simulink model "sign_detector"  (R2026b)
settings: Solver=FixedStepDiscrete  StopTime=5  FixedStep=0.025  EnableMultiTasking=on
values from neighbouring files (symbols this model uses):
  CAN_PERIOD = 0.1    [sign_detector.sldd]
  INFER_PERIOD = 0.05    [sign_detector.sldd]
libraries: raspberrypiAVlib x1
settings Model: DataDictionary=sign_detector.sldd  Creator=don  LastModifiedBy=don
settings SolverCC: PositivePriorityOrder=on
settings OptimizationCC: DifferentSizesBufferReuse=on  EfficientFloat2IntCast=on  EfficientTunableParamExpr=on  EnhancedBackFolding=on  LifeSpan=Inf  MaxStackSize=200000  OptimizationCustomize=off  OptimizeBlockOrder=speed  PassReuseOutputArgsAs=Individual arguments  UseDivisionForNetSlopeComputation=on
settings DebuggingCC: AlgebraicLoopMsg=error  ArtificialAlgebraicLoopMsg=error  AssertControl=DisableAll  BlockPriorityViolationMsg=error  BusObjectLabelMismatch=error  CheckMatrixSingularityMsg=error  InheritedTsInSrcMsg=error  IntegerOverflowMsg=error  IntegerSaturationMsg=error  ModelReferenceDataLoggingMessage=error  ModelReferenceIOMismatchMessage=error  NonBusSignalsTreatedAsBus=error  ParameterPrecisionLossMsg=error  ParameterTunabilityLossMsg=error  ParameterUnderflowMsg=error  ReadBeforeWriteMsg=EnableAllAsError  RootOutportRequireBusObject=error  SFcnCompatibilityMsg=error  SaveWithDisabledLinksMsg=error  SaveWithParameterizedLinksMsg=error  SigSpecEnsureSampleTimeMsg=error  SignalInfNanChecking=error  SignalLabelMismatchMsg=error  SignalRangeChecking=error  SolverPrmCheckMsg=error  StateNameClashWarn=warning  StrictBusMsg=ErrorOnBusTreatedAsVector  TasksWithSamePriorityMsg=error  UnconnectedInputMsg=error  UnconnectedLineMsg=error  UnconnectedOutputMsg=error  UnderSpecifiedDataTypeMsg=error  UniqueDataStoreMsg=error  UnknownTsInhSupMsg=error  UnnecessaryDatatypeConvMsg=warning  VariantConditionMismatch=error  VectorMatrixConversionMsg=error  WriteAfterReadMsg=EnableAllAsError  WriteAfterWriteMsg=EnableAllAsError
settings HardwareCC: ProdHWDeviceType=ARM Compatible->ARM Cortex-A (64-bit)  ProdLargestAtomicFloat=Double  ProdLargestAtomicInteger=LongLong  ProdLongLongMode=on
settings ModelReferenceCC: ModelReferenceNumInstancesAllowed=Single
settings SFSimCC: EnableRuntimeRecursion=off  MATLABDynamicMemAlloc=off
settings RTWCC: BuildConfiguration=Faster Runs  CustomInitializer=ncnn_infer_preload();  Description=Embedded Coder  HardwareBoard=Raspberry Pi (64bit)  PostCodeGenCommand=codertarget.postCodeGenHookCommand(h); pi_postcodegen(buildInfo, string.empty)  SystemTargetFile=ert.tlc  TLCOptions="-aInlineSetEventsForThisBaseRateFcn=TLC_FALSE -aSuppressMultiTaskScheduler=TLC_FALSE  -aRateBasedStepFcn=0"  TargetLang=C++  TemplateMakefile=ert_default_tmf  Toolchain=GNU GCC RPIUtils
settings RTWCC: CustomHeaderCode=|
  | #include <time.h>
  | /* clock_now (Clock Infer, Clock CAN 블록): 단조 시계 [초], Pi 생성 코드에서만 씀 */
  | static inline double mono_time_sec(void)
  | {
  |     struct timespec ts;
  |     clock_gettime(CLOCK_MONOTONIC, &ts);
  |     return (double)ts.tv_sec + (double)ts.tv_nsec * 1e-9;
  | }
  | 
  | /* ncnn_infer.cpp (unit_recognize): 주기 태스크 시작 전에 모델 파일을 읽음 (HIL: 시작 직후 송신 간격 지연 해결) */
  | #ifdef __cplusplus
  | extern "C"
  | #endif
  | int ncnn_infer_preload(void);
settings CodeAppCC: ForceParamTrailComments=on  IgnoreCustomStorageClasses=off  InsertBlockDesc=on  MATLABFcnDesc=on  MATLABSourceComments=on  OperatorAnnotations=on  ReqsInCode=on  SFDataObjDesc=on  SimulinkDataObjDesc=on  StateflowObjectComments=on
settings ERTTargetCC: CastingMode=Standards  CombineSignalStateStructs=on  EnableSignedLeftShifts=off  EnableSignedRightShifts=off  ExtModeIntrfLevel=Level2 - Open  ExtModeMexFile=ext_xcp  ExtModeStaticAlloc=on  GenerateSharedConstants=off  ParenthesesLevel=Standards  PreserveExpressionOrder=on  SubcomponentCodeInterfacePackaging=Nonreusable function  SupportNonFinite=off  SupportVariableSizeSignals=on  SuppressErrorStatus=on  TargetLangStandard=C++11 (ISO)  UtilityFuncGeneration=Shared location

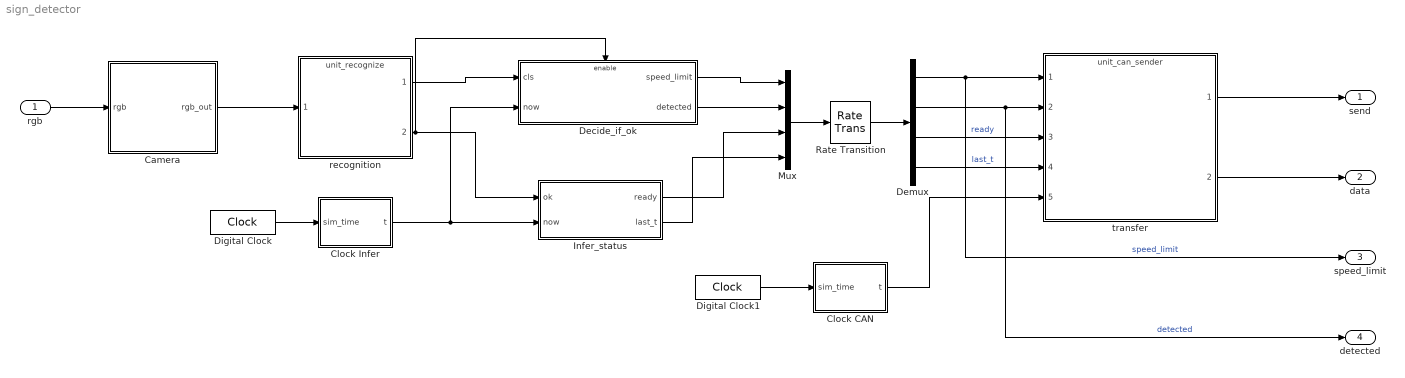
== system sign_detector ==
  rgb : Inport  OutDataTypeStr=uint8  PortDimensions=[480 640 3]  SampleTime=INFER_PERIOD  Interpolate=off
  Camera : Subsystem  Description=rgb 영상 입력 선택 (unit_can_sender의 CAN Tx와 같은 구조)  Variant=on  VariantControlMode=sim codegen switching
  Clock CAN : MATLAB Function  TreatAsAtomicUnit=on
  Clock Infer : MATLAB Function  TreatAsAtomicUnit=on
  Decide_if_ok : Subsystem  Description=|
      | 추론이 성공한 프레임(ok = 1)에서만 unit_decide를 실행.
      | 결과가 없는 프레임은 기록에 넣지 않고, 결과가 STALL_SEC 이상 끊기면 unit_decide가 기록을 비움 (SWR-02, SWR-32)
  Demux : Demux
  Digital Clock : DigitalClock  SampleTime=INFER_PERIOD
  Digital Clock1 : DigitalClock  SampleTime=CAN_PERIOD
  Infer_status : MATLAB Function  TreatAsAtomicUnit=on
  Mux : Mux
  Rate Transition : RateTransition  Description=|  Deterministic=off  OutPortSampleTime=CAN_PERIOD
      | 추론 태스크(0.05 s) -> CAN 태스크(0.1 s).
      | 결정적 전달을 끄고 4개 값을 벡터로 묶어, 추론 스텝이 끝날 때마다 최신 값을 보호 버퍼로 넘김 (추론이 주기를 넘겨도 값이 밀리지 않음, SWR-04, SWR-22)
  recognition : ModelReference  ModelNameDialog=unit_recognize.slx  SimulationMode=Normal  ModelReferenceVersion=1.31
  transfer : ModelReference  ModelNameDialog=unit_can_sender.slx  SimulationMode=Normal  ModelReferenceVersion=1.9
  send : Outport
  data : Outport  Port=2
  speed_limit : Outport  Port=3
  detected : Outport  Port=4
  wires:
  recognition/2 -> Infer_status/1(ok), Decide_if_ok/Enable
  transfer/1 -> send/1
  transfer/2 -> data/1
  Clock Infer/1(t) -> Decide_if_ok/2(now), Infer_status/2(now)
  Clock CAN/1(t) -> transfer/5
  Digital Clock/1 -> Clock Infer/1(sim_time)
  Digital Clock1/1 -> Clock CAN/1(sim_time)
  rgb/1 -> Camera/1(rgb)
  Camera/1(rgb_out) -> recognition/1
  recognition/1 -> Decide_if_ok/1(cls)
  Decide_if_ok/1(speed_limit) -> Mux/1
  Decide_if_ok/2(detected) -> Mux/2
  Infer_status/1(ready) -> Mux/3
  Infer_status/2(last_t) -> Mux/4
  Mux/1 -> Rate Transition/1
  Rate Transition/1 -> Demux/1
  Demux/3 -> transfer/3  "ready"
  Demux/4 -> transfer/4  "last_t"
  Demux/1 -> transfer/1, speed_limit/1  "speed_limit"
  Demux/2 -> transfer/2, detected/1  "detected"

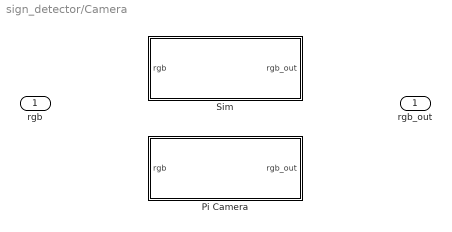
== system sign_detector/Camera ==
  rgb : Inport
  Pi Camera : Subsystem  Description=Pi 생성 코드: 카메라 640x480 RGB -> 480x640x3 (rgb 입력은 쓰지 않음)  VariantControl=(codegen)
  Sim : Subsystem  Description=PC 시뮬레이션과 테스트: 입력포트 rgb(테스트 사진)를 그대로 씀  VariantControl=(sim)
  rgb_out : Outport

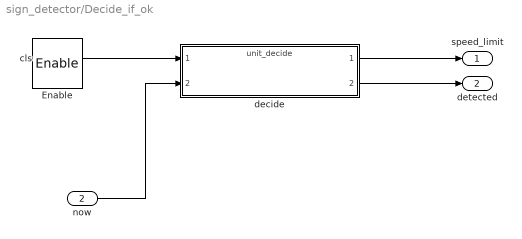
== system sign_detector/Decide_if_ok ==
  cls : Inport
  now : Inport  Port=2
  Enable : EnablePort
  decide : ModelReference  ModelNameDialog=unit_decide.slx  SimulationMode=Normal  ModelReferenceVersion=1.26
  speed_limit : Outport
  detected : Outport  Port=2
  wires:
  cls/1 -> decide/1
  decide/1 -> speed_limit/1
  now/1 -> decide/2
  decide/2 -> detected/1

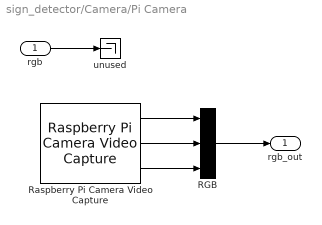
== system sign_detector/Camera/Pi Camera ==
  rgb : Inport
  RGB : Concatenate  NumInputs=3  Mode=Multidimensional array  ConcatenateDimension=3
  Raspberry Pi Camera Video Capture : raspberrypiAVlib/Raspberry Pi Camera Video Capture  CameraNumber=0  Resolution=640x480  CustomResolution=[ 640, 480 ]  PixelFormat=RGB  SampleTime=INFER_PERIOD  HorizontalFlip=off  VerticalFlip=off  ExposureMode=Normal  ExposureCompensation=0.5  MeteringMode=Average  ROI=[ 0.0, 0.0, 1.0, 1.0 ]  Brightness=0.5  Saturation=0.5  Contrast=1  Sharpness=0.5  Rotation=0  AWBMode=Auto
  unused : Terminator
  rgb_out : Outport
  wires:
  rgb/1 -> unused/1
  Raspberry Pi Camera Video Capture/1 -> RGB/1
  Raspberry Pi Camera Video Capture/2 -> RGB/2
  Raspberry Pi Camera Video Capture/3 -> RGB/3
  RGB/1 -> rgb_out/1

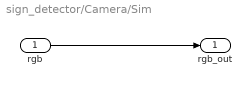
== system sign_detector/Camera/Sim ==
  rgb : Inport
  rgb_out : Outport
  wires:
  rgb/1 -> rgb_out/1

== matlab function sign_detector/Infer_status ==
  data: ok input; ready output; last_t output; now input
function [ready, last_t] = infer_status(ok, now)
% 첫 추론 성공 뒤로 ready = 1 유지 (SWR-34), 마지막으로 성공한 추론 시각 (SWR-32)
persistent r t
if isempty(r)
    r = 0; t = 0;
end
if ok
    r = 1;
    t = now;
end
ready = r;
last_t = t;

== matlab function sign_detector/Clock CAN ==
  data: sim_time input; t output
function t = clock_now(sim_time)
% PC 시뮬레이션: 시뮬레이션 시간 / Pi 생성 코드: 단조 시계 [초]
if coder.target('Rtw')
    t = 0;
    t = coder.ceval('mono_time_sec');
else
    t = sim_time;
end

== matlab function sign_detector/Clock Infer ==
  data: sim_time input; t output
function t = clock_now(sim_time)
% PC 시뮬레이션: 시뮬레이션 시간 / Pi 생성 코드: 단조 시계 [초]
if coder.target('Rtw')
    t = 0;
    t = coder.ceval('mono_time_sec');
else
    t = sim_time;
end
